simulink model "DWPT"  (R2025a)
settings: Solver=VariableStepAuto  StartTime=0.0  StopTime=0.07  FixedStep=Ts  MaxStep=1.0E-7  RelTol=1e-3
InitFcn:
  | f = 85000;
  | Fs = 100000000;       % 100
  | Ts = 1/Fs;          % 步长
  | 
  | 
  | fprintf('周期/Ts = %.10f (应=100)\n', (1/f)/Ts);
  | 
  | 
  | LP1 = 437.3e-6;
  | LP2 = 420.6e-6;
  | LS = 306e-6;
  | LT1 = 98e-6;
  | LT2 = 99.5e-6;
  | 
  | CP1 = 9.03e-9;
  | CP2 = 9.23e-9;
  | 
  | CT1 = 55e-9;
  | CT2 = 54e-9;
  | CS = 12.5e-9;
  | 
  | M1  = 94e-6;
  | M2  = 0e-6;
  | 
  | RP1 = 1.4;
  | RP2 = 1.4;
  | RS = 1.3;
  | 
  | RL = 30;
values from neighbouring files (symbols this model uses):
  M = sum(mu0*sqrt(a*b).*((2-m).*K-2*E)./sqrt(m),'all')    [coil_sizing1200w.m]    (also in coil_sizing250k.m)
undefined symbols (not defined in the file or in its folder): Cp, Lf, Lt
libraries: spsSeriesRLCBranchLib x9, spsCurrentMeasurementLib x8, spsMosfetLib x8, spsRMSLib x7, spsVoltageMeasurementLib x6, spsMeanLib x3, dspfdesign x1, spsDCVoltageSourceLib x1, spsMutualInductanceLib x1, spsUniversalBridgeLib x1, spspowerguiLib x1
settings Model: Creator=yihao  LastModifiedBy=nasa1
settings DataIOCC: ReturnWorkspaceOutputs=off

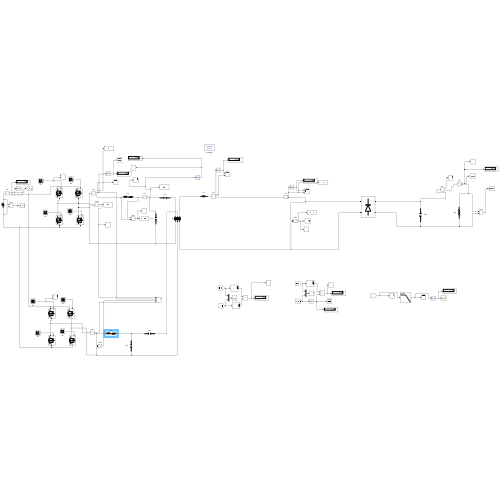
[thumbnail: Simulink's stored preview of the top-level diagram]
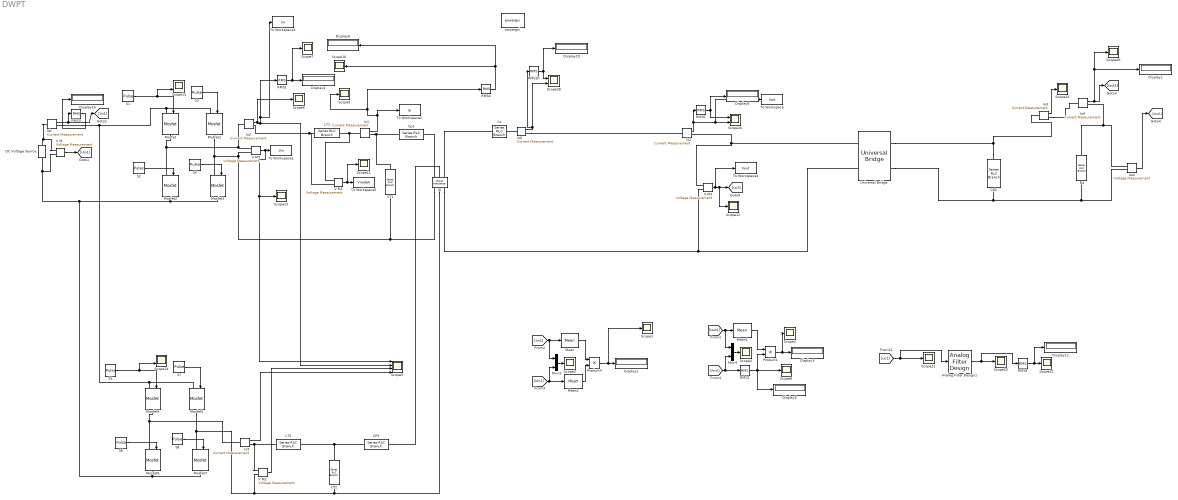
== system DWPT ==
  Analog Filter Design1 : dspfdesign/Analog Filter Design  method=Butterworth  filttype=Lowpass  N=8  Wlo=85000*2*pi  Whi=80  Rp=2  Rs=40
  CP2 : spsSeriesRLCBranchLib/Series RLC Branch  LConnTagsString=__new0  RConnTagsString=__new0  BranchType=C  Resistance=0.1  Inductance=1e-3  SetiL0=off  InitialCurrent=0  Capacitance=CP2  Setx0=off  InitialVoltage=0  Measurements=None
  CT1 : spsSeriesRLCBranchLib/Series RLC Branch  LConnTagsString=__new0  RConnTagsString=__new0  BranchType=C  Resistance=0.1  Inductance=1e-3  SetiL0=off  InitialCurrent=0  Capacitance=CT1  Setx0=off  InitialVoltage=0  Measurements=None
  CT2 : spsSeriesRLCBranchLib/Series RLC Branch  LConnTagsString=__new0  RConnTagsString=__new0  BranchType=C  Resistance=0.1  Inductance=1e-3  SetiL0=off  InitialCurrent=0  Capacitance=CT2  Setx0=off  InitialVoltage=0  Measurements=None
  Cd2 : spsSeriesRLCBranchLib/Series RLC Branch  LConnTagsString=__new0  RConnTagsString=__new0  BranchType=C  Resistance=0.01  Inductance=1e-3  SetiL0=off  InitialCurrent=0  Capacitance=470e-6  Setx0=off  InitialVoltage=100  Measurements=None
  Cp1 : spsSeriesRLCBranchLib/Series RLC Branch  LConnTagsString=__new0  RConnTagsString=__new0  BranchType=C  Resistance=0.1  Inductance=1e-3  SetiL0=off  InitialCurrent=0  Capacitance=CP1  Setx0=off  InitialVoltage=0  Measurements=None
  Cs : spsSeriesRLCBranchLib/Series RLC Branch  LConnTagsString=__new0  RConnTagsString=__new0  BranchType=C  Resistance=0.01  Inductance=1e-3  SetiL0=off  InitialCurrent=0  Capacitance=CS  Setx0=off  InitialVoltage=0  Measurements=None
  DC Voltage Source : spsDCVoltageSourceLib/DC Voltage Source  Amplitude=50  Measurements=None
  Display{1..6,8,12,16,19} (10 alike) : Display
  Idc : spsCurrentMeasurementLib/Current Measurement  PhasorSimulation=off  OutputType=Complex  PSBequivalent=0
  Io{1..6} (6 alike) : spsCurrentMeasurementLib/Current Measurement  PhasorSimulation=off  OutputType=Complex  PSBequivalent=0
  Is2 : spsCurrentMeasurementLib/Current Measurement  PhasorSimulation=off  OutputType=Complex  PSBequivalent=0
  LT1 : spsSeriesRLCBranchLib/Series RLC Branch  LConnTagsString=__new0  RConnTagsString=__new0  BranchType=RL  Resistance=0.1  Inductance=LT1  SetiL0=off  InitialCurrent=0  Capacitance=Cp  Setx0=off  InitialVoltage=0  Measurements=None
  LT2 : spsSeriesRLCBranchLib/Series RLC Branch  LConnTagsString=__new0  RConnTagsString=__new0  BranchType=RL  Resistance=0.1  Inductance=LT2  SetiL0=off  InitialCurrent=0  Capacitance=Cp  Setx0=off  InitialVoltage=0  Measurements=None
  M : spsMutualInductanceLib/Mutual Inductance  LConnTagsString=a|b|c  RConnTagsString=A|B|C  TypeOfMutual=Generalized mutual inductance  NumberOfWindings=3  SelfImpedance1=[0.06 Lf]  SelfImpedance2=[0.06 Lt]  ThreeWindings=off  SelfImpedance3=[ 1.1 1.1e-03]  MutualImpedance=[0 M]  InductanceMatrix=[LP1 0 M1; 0 LP2 M2;M1 M2 LS]  ResistanceMatrix="[RP1  0 0; 0  RP2 0; 0 0 RS]"  Measurements=None
  Mean : spsMeanLib/Mean  Freq=f/100  Vinit=0  Ts=0
  Mean1 : spsMeanLib/Mean  Freq=f  Vinit=0  Ts=0
  Mean2 : spsMeanLib/Mean  Freq=f/100  Vinit=0  Ts=0
  Mosfet{,1..7} (8 alike) : spsMosfetLib/Mosfet  Ron=0.09  Lon=0  Rd=0.01  Vfd=3.3  IC=0  Rs=1e5  Cs=inf  Measurements=off
  Mux3 : Mux  Inputs=2
  Mux4 : Mux  Inputs=2
  Product1 : Product
  Product4 : Product
  R4 : spsSeriesRLCBranchLib/Series RLC Branch  LConnTagsString=__new0  RConnTagsString=__new0  BranchType=R  Resistance=30  Inductance=1e-6  SetiL0=off  InitialCurrent=0  Capacitance=Cp  Setx0=off  InitialVoltage=0  Measurements=None
  RMS{1,3..4,6,8,10} (6 alike) : spsRMSLib/RMS  TrueRMS=on  Freq=f/100  RMSInit=0  Ts=0
  RMS2 : spsRMSLib/RMS  TrueRMS=on  Freq=f/100  RMSInit=120  Ts=0
  S{1,4..5,8} (4 alike) : DiscretePulseGenerator  PulseType=Time based  Period=1/f  PulseWidth=49.5
  S{2..3,6..7} (4 alike) : DiscretePulseGenerator  PulseType=Time based  Period=1/f  PulseWidth=49.5  PhaseDelay=1/2/f
  Scope{1..4,6..12,20..24,26} (17 alike) : Scope
      Scope1 settings: ActiveDisplayYMinimum=-49.10464  ActiveDisplayYMaximum=441.94179  DataLoggingSaveFormat=Array
      Scope10 settings: ActiveDisplayYMinimum=-0.71464  ActiveDisplayYMaximum=6.43176  DataLoggingVariableName=ScopeData2  DataLoggingSaveFormat=Array
      Scope11 settings: ActiveDisplayYMinimum=-10.18584  ActiveDisplayYMaximum=11.18954  DataLoggingSaveFormat=Array
      Scope12 settings: ActiveDisplayYMinimum=-124.85082  ActiveDisplayYMaximum=124.97825  DataLoggingVariableName=ScopeData4  DataLoggingSaveFormat=Array
      Scope2 settings: ActiveDisplayYMinimum=-3.3359920538155139  ActiveDisplayYMaximum=30.023928484339635  DataLoggingVariableName=ScopeData12  DataLoggingSaveFormat=Array
      Scope20 settings: ActiveDisplayYMinimum=-998.97593  ActiveDisplayYMaximum=1003.83836  DataLoggingVariableName=ScopeData13  DataLoggingSaveFormat=Array
      Scope21 settings: ActiveDisplayYMinimum=-1098.42082  ActiveDisplayYMaximum=1097.9597  DataLoggingVariableName=ScopeData14  DataLoggingSaveFormat=Array
      Scope22 settings: ActiveDisplayYMinimum=-0.08617  ActiveDisplayYMaximum=0.77556  DataLoggingVariableName=ScopeData15  DataLoggingSaveFormat=Array
      Scope23 settings: ActiveDisplayYMinimum=-126.90541  ActiveDisplayYMaximum=126.90651  DataLoggingVariableName=ScopeData16  DataLoggingSaveFormat=Array
      Scope24 settings: ActiveDisplayYMinimum=-0.06956  ActiveDisplayYMaximum=0.62607  DataLoggingSaveFormat=Array
      Scope26 settings: ActiveDisplayYMinimum=-0.31456  ActiveDisplayYMaximum=2.83101  DataLoggingVariableName=ScopeData2  DataLoggingSaveFormat=Array
      Scope3 settings: ActiveDisplayYMinimum=-3742.24205  ActiveDisplayYMaximum=32139.40337  DataLoggingVariableName=ScopeData23  DataLoggingSaveFormat=Array
      Scope4 settings: ActiveDisplayYMinimum=-3.3830504056400548  ActiveDisplayYMaximum=30.4474536507605  DataLoggingVariableName=ScopeData27  DataLoggingSaveFormat=Array
      Scope6 settings: ActiveDisplayYMinimum=-10.18584  ActiveDisplayYMaximum=11.18954  DataLoggingVariableName=ScopeData29  DataLoggingSaveFormat=Array
      Scope7 settings: ActiveDisplayYMinimum=41.35748  ActiveDisplayYMaximum=44.91904  DataLoggingVariableName=ScopeData30  DataLoggingSaveFormat=Array
      Scope8 settings: ActiveDisplayYMinimum=-10.89533  ActiveDisplayYMaximum=134.54393  DataLoggingVariableName=ScopeData31  DataLoggingSaveFormat=Array
      Scope9 settings: ActiveDisplayYMinimum=-11.00674  ActiveDisplayYMaximum=11.77758  DataLoggingSaveFormat=Array
  Scope{13..14,16,28} (4 alike) : Scope  NumInputPorts=2
      Scope13 settings: ActiveDisplayYMinimum=-12.75848  ActiveDisplayYMaximum=112.74941  DataLoggingVariableName=ScopeData5  DataLoggingSaveFormat=Array
      Scope14 settings: ActiveDisplayYMinimum=-12.75848  ActiveDisplayYMaximum=112.74941  DataLoggingVariableName=ScopeData3  DataLoggingSaveFormat=Array
      Scope16 settings: ActiveDisplayYMinimum=-5.8521517419594016  ActiveDisplayYMaximum=5.8917781570828591  DataLoggingVariableName=ScopeData8  DataLoggingSaveFormat=Array
      Scope28 settings: ActiveDisplayYMinimum=-4.84326  ActiveDisplayYMaximum=4.41106  DataLoggingVariableName=ScopeData21  DataLoggingSaveFormat=Array
  Scope5 : Scope  NumInputPorts=4
      settings: ActiveDisplayYMinimum=-71.017946366553787  ActiveDisplayYMaximum=71.042097514829976  DataLoggingVariableName=ScopeData28  DataLoggingSaveFormat=Array
  To Workspace : ToWorkspace  VariableName=Iout  SaveFormat=Structure With Time  SampleTime=-1
  To Workspace1 : ToWorkspace  VariableName=Vin  SaveFormat=Structure With Time  SampleTime=-1
  To Workspace2 : ToWorkspace  VariableName=Ip  SaveFormat=Structure With Time  SampleTime=-1
  To Workspace3 : ToWorkspace  VariableName=Iin  SaveFormat=Structure With Time  SampleTime=-1
  To Workspace4 : ToWorkspace  VariableName=Vout  SaveFormat=Structure With Time  SampleTime=-1
  To Workspace5 : ToWorkspace  VariableName=VnodeA  SaveFormat=Structure With Time  SampleTime=-1
  Universal Bridge : spsUniversalBridgeLib/Universal Bridge  Arms=2  SnubberResistance=1e5  SnubberCapacitance=inf  Device=Diodes  Ron=0.03  Lon=0  ForwardVoltages="[  0  0  ]"  ForwardVoltage=1.5  GTOparameters=[ 10e-6 , 20e-6 ]  IGBTparameters=[ 1e-6 , 2e-6 ]  Measurements=None  Measurements_2=None  converterType=Rectifier
  Uo2 : spsVoltageMeasurementLib/Voltage Measurement  PhasorSimulation=off  OutputType=Complex  PSBequivalent=0
  V M{,1..3,5} (5 alike) : spsVoltageMeasurementLib/Voltage Measurement  PhasorSimulation=off  OutputType=Complex  PSBequivalent=0
  powergui : spspowerguiLib/powergui  Priority=1  SimulationMode=Discrete  SampleTime=1e-7  frequency=60  Iterations=50  frequencyindice=0  Pbase=100e6  ErrMax=1e-4  UnitsV=kV  UnitsW=MW  buscounter=0  FunctionMessages=off  echomessages=off  EnableUseOfTLC=off  CurrentSourceSwitches=off  DisableSnubberDevices=off  DisableRonSwitches=off  DisableVfSwitches=off  DisplayEquations=off  AutomaticDiscreteSolvers=off  SolverType=Tustin/Backward Euler (TBE)  Interpol=off  ExternalGateDelay=off  methode=off  Ts=100  x0status=blocks  SPID=on  SwTol=0  HookPort=off  NonlinearTolerance=1e-4  nMaxIteration=100  ContinueOnMaxIteration=off  RestoreLinks=warning  ResistiveCurrentMeasurement=off  Frange=[0:2:500]  Ylog=off  Xlog=on  ShowGrid=off  save=off  variable=ZData  structure=Is2  ZoomFFT=off  StartTime=0.1  cycles=5  DisplayStyle=1  fundamental=85000  FreqAxis=off  MaxFrequency=100000  frequencyindicesteady=1  RmsSteady=1  display=off
  wires:
  Is2/1 -> To Workspace/1, Scope16/2, RMS6/1
  Io6/1 -> Scope28/2, RMS10/1
  [Uin1] -> Mean2/1, Mux3/2
  V M5/1 -> To Workspace1/1, Scope5/1, Scope23/1
  [Uout1] -> RMS2/1, Mux4/2
  RMS4/1 -> Display6/1, Scope10/1
  Mean/1 -> Product4/1
  Idc/1 -> RMS3/1, [Iin1]
  V M3/1 -> To Workspace4/1, Scope12/1, [uc2]
  Mean1/1 -> Product1/1
  Io2/1 -> Scope5/2, To Workspace3/1, RMS1/1, Scope6/1
  [Iin1] -> Mean/1, Mux3/1
  S2/1 -> Mosfet2/1
  RMS2/1 -> Display5/1, Scope8/1, Product1/2
  Mux4/1 -> Scope4/1
  Mean2/1 -> Product4/2
  [uc2] -> Analog Filter Design1/1, Scope21/1
  Product1/1 -> Scope2/1, Display3/1
  S4/1 -> Mosfet3/1
  V M/1 -> [Uin1]
  Mux3/1 -> Scope3/1
  [Iout1] -> Mean1/1, Mux4/1
  RMS8/1 -> Display12/1, Scope22/1
  RMS1/1 -> Display4/1, Scope7/1
  Analog Filter Design1/1 -> RMS8/1, Scope20/1
  S1/1 -> Scope13/2, Mosfet/1
  RMS6/1 -> Scope16/1, Display8/1
  Product4/1 -> Scope1/1, Display2/1
  RMS10/1 -> Scope28/1, Display19/1
  S3/1 -> Mosfet1/1
  Io1/1 -> To Workspace2/1, RMS4/1, Scope9/1
  RMS3/1 -> Display16/1
  V M1/1 -> Scope11/1, To Workspace5/1
  Uo2/1 -> [Uout1]
  Io4/1 -> Display1/1, Scope26/1, [Iout1]
  Io3/1 -> Scope24/1
  V M2/1 -> Scope5/3
  Io5/1 -> Scope5/4
  S8/1 -> Mosfet7/1
  S5/1 -> Scope14/2, Mosfet4/1
  S6/1 -> Mosfet6/1
  S7/1 -> Mosfet5/1
  connections:
  Mosfet6/RConn1 -- DC Voltage Source/LConn1 -- V M/LConn2 -- Mosfet3/RConn1 -- Mosfet2/RConn1 -- Mosfet7/RConn1
  V M5/LConn1 -- Mosfet/RConn1 -- Mosfet2/LConn1 -- Io2/LConn1
  Idc/LConn1 -- DC Voltage Source/RConn1 -- V M/LConn1
  V M3/LConn1 -- Universal Bridge/LConn1 -- Is2/RConn1
  Io6/RConn1 -- Is2/LConn1
  Mosfet5/LConn1 -- Idc/RConn1 -- Mosfet/LConn1 -- Mosfet1/LConn1 -- Mosfet4/LConn1
  Io6/LConn1 -- Cs/LConn1
  Mosfet1/RConn1 -- Mosfet3/LConn1 -- CT1/RConn1 -- M/RConn1 -- V M5/LConn2
  M/LConn3 -- Cs/RConn1
  LT1/RConn1 -- V M1/LConn2 -- Io2/RConn1
  Io1/RConn1 -- CT1/LConn1 -- Cp1/RConn1
  Io1/LConn1 -- V M1/LConn1 -- LT1/LConn1
  Universal Bridge/LConn2 -- M/RConn3 -- V M3/LConn2
  Uo2/LConn1 -- R4/LConn1 -- Io4/RConn1
  Io3/RConn1 -- Io4/LConn1
  R4/RConn1 -- Uo2/LConn2 -- Cd2/RConn1 -- Universal Bridge/RConn2
  Cd2/LConn1 -- Io3/LConn1 -- Universal Bridge/RConn1
  CT2/LConn1 -- CP2/RConn1 -- LT2/LConn1
  CP2/LConn1 -- M/LConn2
  M/LConn1 -- Cp1/LConn1
  V M2/LConn1 -- Io5/RConn1 -- LT2/RConn1
  Mosfet6/LConn1 -- Io5/LConn1 -- Mosfet4/RConn1
  Mosfet7/LConn1 -- V M2/LConn2 -- M/RConn2 -- CT2/RConn1 -- Mosfet5/RConn1
